simulink model "PVonGrid_patched"  (R2025a)
settings: Solver=VariableStepAuto  StartTime=0.0  StopTime=2.0  RelTol=1e-3
PreLoadFcn:
  | % Parameter basis-watt yang menghasilkan Gambar 6 pada naskah.
  | % Sama persis dengan matlab/siapkan_workspace.m. JANGAN pakai
  | % init_VIC.m: nilainya set per-unit lama dan menghasilkan respons
  | % yang sama sekali berbeda.
  | f0 = 50;  Kw = 1;  H = 4;  Ts = 1e-5;
  | num_Tdi = 1;     den_Tdi    = [0.01 1];
  | num_Tri = 1;     den_Tri    = [0.01 1];
  | num_filter = 1;  den_filter = [0.02 1];
  | Dv = 20000;      Kiv = 632;
  | clear Prated R T_filter Tdi Tri VIC_max VIC_min
undefined symbols (not defined in the file): DiscIntNeverNeededParam, Down, Ion, Lithium, Up
libraries: spsSeriesRLCBranchLib x15, mcbeeMathTransformLib x8, spsIGBTDiodeLib x5, spsCurrentMeasurementLib x4, spsVoltageMeasurementLib x4, slpidlib x3, spsThreePhaseVIMeasurementLib x3, spsMosfetLib x2, spsDiodeLib x2, spsGroundLib x2, spsUniversalBridgeLib x2, spsPower3phInstantaneousLib x2
(part 2 of 2)

== matlab function PVonGrid_patched/MPPT Controller/MPPT Algorithm ==
  settings: updateMethod=DISCRETE
  data: V input; Iref output; I input
%Incremental Conductance Algorithm for PV
function Iref = MPPT_INC(V,I)

Irefinit = 0;
Irefmax = 70;
Irefmin = 0;
deltaIref = 0.0008;

persistent Vold Iold Irefold

if isempty(Vold)
    Vold = 0;
    Iold = 0;
    Irefold = Irefinit;
end

dV = V - Vold;
dI = I - Iold;

if dV == 0
    if dI == 0
        Iref = Irefold;
    elseif dI > 0
        Iref = Irefold + (deltaIref);
    else
        Iref = Irefold - (deltaIref);
    end
    else
    if dI/dV == -I/V
        Iref = Irefold;
    elseif dI/dV > -I/V
        Iref = Irefold - (deltaIref);
    else
        Iref = Irefold + (deltaIref);
    end
end

if Iref >= Irefmax || Iref <= Irefmin
    Iref = Irefold;
end

Irefold = Iref;
Vold = V;
Iold = I;
